simulink model "rlc_series"  (R2025b)
settings: Solver=ode45  StartTime=0.0  StopTime=p.stopTime  MaxStep=p.sampleTime  RelTol=1e-8  AbsTol=1e-10
model workspace (MAT data in the model file):
  p.R = 12
  p.L = 0.008
  p.C = 1.2e-05
  p.sourceVoltage = 5
  p.sourceTime = 0.001
  p.secondStepVoltage = 0.75
  p.secondStepTime = 0.00661
  p.sampleTime = 2e-06
  p.stopTime = 0.012812
values from neighbouring files (symbols this model uses):
  p = project_parameters()    [run_demo.m]
settings Model: Creator=LENOVO  LastModifiedBy=LENOVO

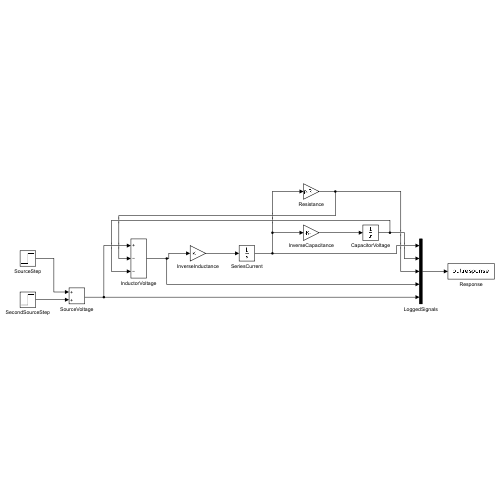
[thumbnail: Simulink's stored preview of the top-level diagram]
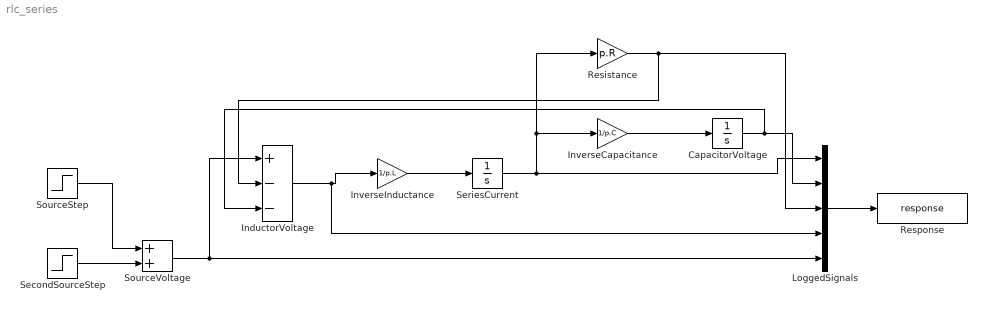
== system rlc_series ==
  CapacitorVoltage : Integrator
  InductorVoltage : Sum  Inputs=+--
  InverseCapacitance : Gain  Gain=1/p.C
  InverseInductance : Gain  Gain=1/p.L
  LoggedSignals : Mux  Inputs=5
  Resistance : Gain  Gain=p.R
  Response : ToWorkspace  VariableName=response  SaveFormat=Timeseries  SampleTime=-1
  SecondSourceStep : Step  Time=p.secondStepTime  After=p.secondStepVoltage  SampleTime=0
  SeriesCurrent : Integrator
  SourceStep : Step  Time=p.sourceTime  After=p.sourceVoltage  SampleTime=0
  SourceVoltage : Sum
  wires:
  LoggedSignals/1 -> Response/1
  InverseCapacitance/1 -> CapacitorVoltage/1
  SeriesCurrent/1 -> Resistance/1, InverseCapacitance/1, LoggedSignals/1
  InverseInductance/1 -> SeriesCurrent/1
  InductorVoltage/1 -> InverseInductance/1, LoggedSignals/4
  CapacitorVoltage/1 -> InductorVoltage/3, LoggedSignals/2
  Resistance/1 -> LoggedSignals/3, InductorVoltage/2
  SourceVoltage/1 -> InductorVoltage/1, LoggedSignals/5
  SecondSourceStep/1 -> SourceVoltage/2
  SourceStep/1 -> SourceVoltage/1
